simulink model "decodeur_hamming_slx"  (R2023b)
settings: Solver=FixedStepDiscrete  StartTime=0.0  StopTime=Tstop  FixedStep=1  RelTol=1e-3
settings Model: Creator=e2604176  LastModifiedBy=e2604176
settings OptimizationCC: BooleanDataType=off

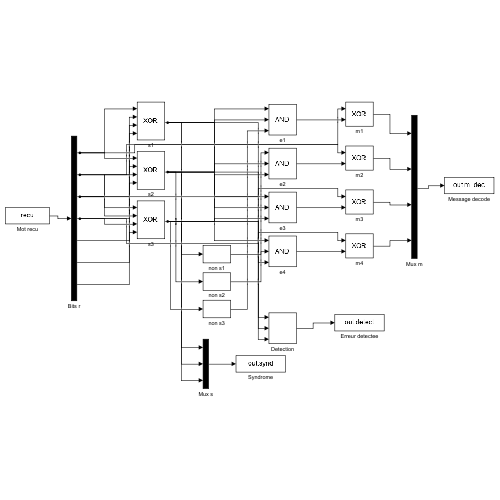
[thumbnail: Simulink's stored preview of the top-level diagram]
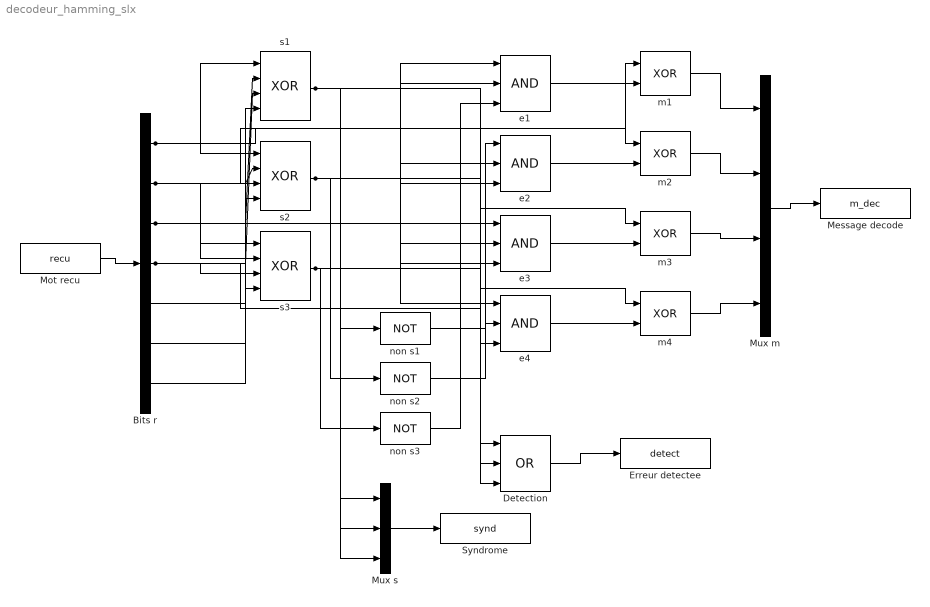
== system decodeur_hamming_slx ==
  Bits r : Demux  Outputs=7
  Detection : Logic  Operator=OR  Inputs=3  AllPortsSameDT=off  OutDataTypeStr=boolean
  Erreur detectee : ToWorkspace  VariableName=detect  SampleTime=-1
  Message decode : ToWorkspace  VariableName=m_dec  SampleTime=-1
  Mot recu : FromWorkspace  VariableName=recu  SampleTime=1  Interpolate=off  OutputAfterFinalValue=Setting to zero
  Mux m : Mux
  Mux s : Mux  Inputs=3
  Syndrome : ToWorkspace  VariableName=synd  SampleTime=-1
  e{1..4} (4 alike) : Logic  Inputs=3  AllPortsSameDT=off  OutDataTypeStr=boolean
  m{1..4} (4 alike) : Logic  Operator=XOR  AllPortsSameDT=off  OutDataTypeStr=boolean
  non s1 : Logic  Operator=NOT  Inputs=1  AllPortsSameDT=off  OutDataTypeStr=boolean
  non s2 : Logic  Operator=NOT  Inputs=1  AllPortsSameDT=off  OutDataTypeStr=boolean
  non s3 : Logic  Operator=NOT  Inputs=1  AllPortsSameDT=off  OutDataTypeStr=boolean
  s1 : Logic  Operator=XOR  Inputs=4  AllPortsSameDT=off  OutDataTypeStr=boolean
  s2 : Logic  Operator=XOR  Inputs=4  AllPortsSameDT=off  OutDataTypeStr=boolean
  s3 : Logic  Operator=XOR  Inputs=4  AllPortsSameDT=off  OutDataTypeStr=boolean
  wires:
  Mot recu/1 -> Bits r/1
  Bits r/1 -> s1/1, s2/1, m1/1
  Bits r/3 -> s1/2, s2/3, s3/2, m3/1
  Bits r/4 -> s1/3, s3/3, m4/1
  Bits r/5 -> s1/4
  Bits r/2 -> s2/2, s3/1, m2/1
  Bits r/6 -> s2/4
  Bits r/7 -> s3/4
  s1/1 -> non s1/1, e1/1, e3/1, e4/1, Detection/1, Mux s/1
  s2/1 -> non s2/1, e1/2, e2/2, e3/2, Detection/2, Mux s/2
  s3/1 -> non s3/1, e2/3, e3/3, e4/3, Detection/3, Mux s/3
  non s3/1 -> e1/3
  non s1/1 -> e2/1
  non s2/1 -> e4/2
  e1/1 -> m1/2
  e2/1 -> m2/2
  e3/1 -> m3/2
  e4/1 -> m4/2
  Detection/1 -> Erreur detectee/1
  m1/1 -> Mux m/1
  m2/1 -> Mux m/2
  m3/1 -> Mux m/3
  m4/1 -> Mux m/4
  Mux m/1 -> Message decode/1
  Mux s/1 -> Syndrome/1
